simulink model "Quadcopter_2DoF_Model_7_b"  (R2025b)
settings: Solver=ode23t  StartTime=0.0  StopTime=T_mis  FixedStep=0.02  MaxStep=0.001  RelTol=1e-3
InitFcn:
  | % Make sure MATLAB can find the model folder and the battery data folder
  | modelDir = fileparts(get_param(bdroot, 'FileName'));
  | addpath(modelDir);  % finds mission_config.m
  | addpath(fullfile(modelDir, '..', 'Battery_data', 'output')); % finds hppc_params.mat
  | 
  | 
  | %Quadcopter parameters
  | Jyy = 5.343596e-5; %Mass moment of inertia about yB(kg.m^2)
  | Jxx = 5.473766e-5;%Mass moment of inertia about xB(kg.m^2)
  | Jzz = 9.8934e-5;%Mass moment of inertia about zB(kg.m^2)
  | m = 0.1207; %Total mass of the quadcopter (kg)
  | g = 9.81; %gravitational acceleration
  | k_f = 7.22e-8; %thrust coefficient
  | k_tau = 5.11e-10; %torque coefficient. smaller than kf
  | l = 0.05433; %Arm length, COM to each motor shaft
  | 
  | %Battery parameters
  | if ~exist('soc0', 'var'), soc0 = 1; end
  | load('hppc_params.mat', 'soc_grid', 'tables');
  | 
  | idx      = 1:5:101; % every 5% SOC, 21 points
  | SOC_vec  = soc_grid(idx)'; % 0, 0.05, ... 1
  | V0_vec   = tables.OCV(idx)';
  | R0_vec   = tables.R0(idx)'  / 1000;
  | R1_vec   = tables.R1(idx)'  / 1000;
  | tau1_vec = R1_vec .* tables.C1(idx)';
  | 
  | %Mission parameters
  | mis = mission_config('fast_move', false);
  | t_mis = mis.t;
  | z_ref = mis.z;
  | x_ref = mis.x;
  | T_mis = mis.T;
values from neighbouring files (symbols this model uses):
  soc_grid = [0 0.01 0.02 0.03 0.04 0.05 0.06 0.07 0.08 0.09 0.1 0.11 ... (101 elements, 101x1)]    [hppc_params.mat]
  tables =     [hppc_params.mat]
libraries: fl_lib x4, slpidlib x3, nesl_utility x3, simulink x3
settings Model: Creator=Haaniya  LastModifiedBy=Haaniya
settings DataIOCC: ReturnWorkspaceOutputs=off

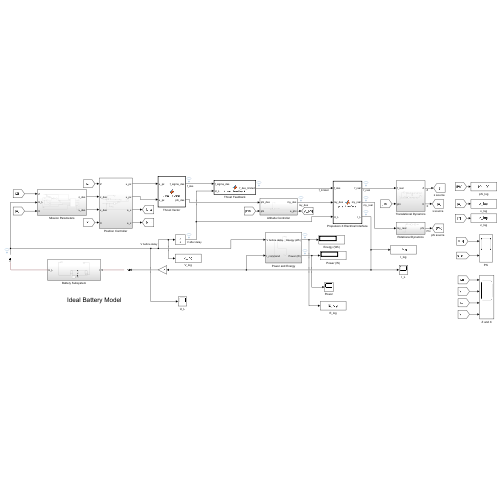
[thumbnail: Simulink's stored preview of the top-level diagram]
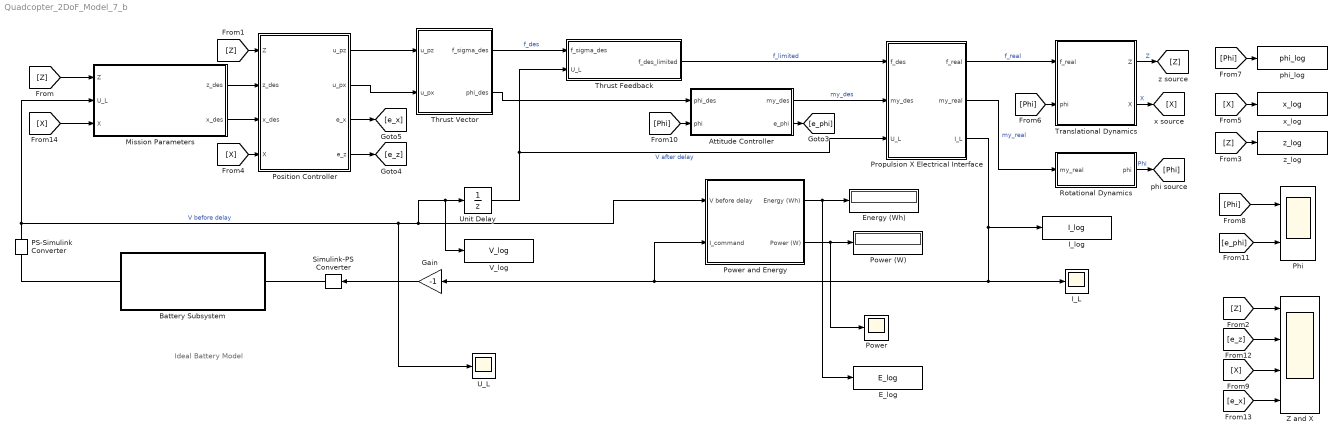
== system Quadcopter_2DoF_Model_7_b ==
  note: Ideal Battery Model
  Attitude Controller : Subsystem
  Battery Subsystem : Subsystem
  E_log : ToWorkspace  VariableName=E_log  SaveFormat=Timeseries  SampleTime=-1
  Energy (Wh) : Display
  Gain : Gain  Gain=-1
  I_L : Scope
      settings: ActiveDisplayYMinimum=-1  ActiveDisplayYMaximum=1  DataLoggingVariableName=ScopeData5
  I_log : ToWorkspace  VariableName=I_log  SaveFormat=Timeseries  SampleTime=-1
  Mission Parameters : Subsystem
  PS-Simulink Converter : nesl_utility/PS-Simulink Converter  PhysicalDomain=network_engine_domain  SubClassName=ps_output  LeftPortType=input  RightPortType=output  PseudoPeriodic=off  Frequencies=[]  VectorFormat=inherit  Unit=inherit  AffineConversion=off
  Phi : Scope  NumInputPorts=2
      settings: ActiveDisplayYMinimum=-0.256680900083002  ActiveDisplayYMaximum=0.30893996648524746
  Position Controller : Subsystem
  Power : Scope
      settings: ActiveDisplayYMinimum=-1  ActiveDisplayYMaximum=1
  Power (W) : Display
  Power and Energy : Subsystem
  Propulsion X Electrical Interface : MATLAB Function  TreatAsAtomicUnit=on
  Rotational Dynamics : Subsystem
  Simulink-PS Converter : nesl_utility/Simulink-PS Converter  PhysicalDomain=network_engine_domain  SubClassName=ps_input  LeftPortType=input  RightPortType=output  PseudoPeriodic=off  Frequencies=[]  NoiseDistribution=none  NoiseParameters=[]  Unit=1  AffineConversion=off  FilteringAndDerivatives=provide  SimscapeFilterOrder=1  InputFilterTimeConstant=0.001  UdotUserProvided=0
  Thrust Feedback : MATLAB Function  TreatAsAtomicUnit=on
  Thrust Vector : MATLAB Function  TreatAsAtomicUnit=on
  Translational Dynamics : Subsystem
  U_L : Scope
      settings: ActiveDisplayYMinimum=-1  ActiveDisplayYMaximum=1  DataLoggingVariableName=ScopeData4
  Unit Delay : UnitDelay  InitialCondition=12.6  SampleTime=-1  HasFrameUpgradeWarning=on
  V_log : ToWorkspace  VariableName=V_log  SaveFormat=Timeseries  SampleTime=-1
  Z and X : Scope  NumInputPorts=4
      settings: ActiveDisplayYMinimum=-2.8823289084594785  ActiveDisplayYMaximum=7.6709964500964789  DataLoggingVariableName=ScopeData2
  phi_log : ToWorkspace  VariableName=phi_log  SaveFormat=Timeseries  SampleTime=0.02
  x_log : ToWorkspace  VariableName=x_log  SaveFormat=Timeseries  SampleTime=0.02
  z_log : ToWorkspace  VariableName=z_log  SaveFormat=Timeseries  SampleTime=0.02
  wires:
  Position Controller/2(u_px) -> Thrust Vector/2(u_px)
  Position Controller/1(u_pz) -> Thrust Vector/1(u_pz)
  Thrust Vector/2(phi_des) -> Attitude Controller/1(phi_des)
  Propulsion X Electrical Interface/2(my_real) -> Rotational Dynamics/1(my_real)  "my_real"
  Unit Delay/1 -> Thrust Feedback/2(U_L), Propulsion X Electrical Interface/3(U_L)  "V after delay"
  PS-Simulink Converter/1 -> Mission Parameters/2(U_L), U_L/1, V_log/1, Unit Delay/1, Power and Energy/1(V before delay)  "V before delay"
  Gain/1 -> Simulink-PS Converter/1
  Propulsion X Electrical Interface/3(I_L) -> I_L/1, Power and Energy/2(I_command), Gain/1, I_log/1
  Propulsion X Electrical Interface/1(f_real) -> Translational Dynamics/1(f_real)  "f_real"
  Attitude Controller/1(my_des) -> Propulsion X Electrical Interface/2(my_des)  "my_des"
  Thrust Vector/1(f_sigma_des) -> Thrust Feedback/1(f_sigma_des)  "f_des"
  Thrust Feedback/1(f_des_limited) -> Propulsion X Electrical Interface/1(f_des)  "f_limited"
  Mission Parameters/1(z_des) -> Position Controller/2(z_des)
  Mission Parameters/2(x_des) -> Position Controller/3(x_des)
  [Z] -> Mission Parameters/1(Z)
  [Z] -> Position Controller/1(Z)
  [Z] -> Z and X/1
  Translational Dynamics/1(Z) -> [Z]  "Z"
  [Z] -> z_log/1
  [X] -> Position Controller/4(X)
  [X] -> x_log/1
  Translational Dynamics/2(X) -> [X]  "X"
  [Phi] -> Translational Dynamics/2(phi)
  [Phi] -> phi_log/1
  [Phi] -> Phi/1
  [X] -> Z and X/3
  [Phi] -> Attitude Controller/2(phi)
  Rotational Dynamics/1(phi) -> [Phi]  "Phi"
  [e_phi] -> Phi/2
  [e_z] -> Z and X/2
  [e_x] -> Z and X/4
  Attitude Controller/2(e_phi) -> [e_phi]
  Position Controller/4(e_z) -> [e_z]
  Position Controller/3(e_x) -> [e_x]
  Power and Energy/1(Energy (Wh)) -> E_log/1, Energy (Wh)/1
  Power and Energy/2(Power (W)) -> Power/1, Power (W)/1
  [X] -> Mission Parameters/3(X)
  connections:
  Battery Subsystem/LConn1 -- PS-Simulink Converter/LConn1
  Simulink-PS Converter/RConn1 -- Battery Subsystem/RConn1

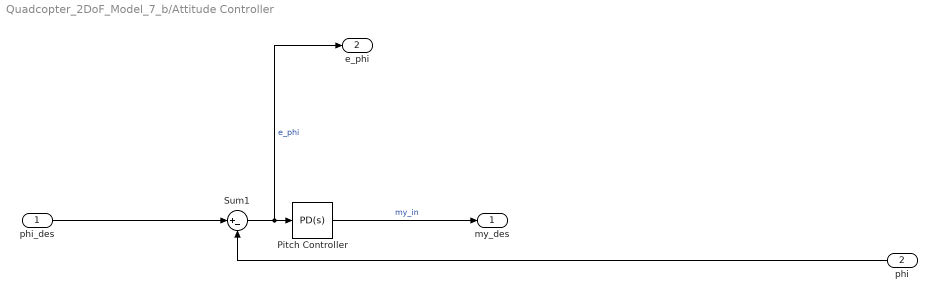
== system Quadcopter_2DoF_Model_7_b/Attitude Controller ==
  phi_des : Inport
  phi : Inport  Port=2
  Pitch Controller : slpidlib/PID Controller  Controller=PD  Form=Parallel  TimeDomain=Continuous-time  UseExternalTs=off  SampleTime=-1  IntegratorMethod=Forward Euler  FilterMethod=Forward Euler  ControllerParametersSource=internal  P=0.000320082486755336  I=1  UseKiTs=off  D=0.000451023727668426  UseExternalDerivativeSource=off  N=23.8205218545542  UseFilter=on  TunerSelectOption=Transfer Function Based (PID Tuner App)  InitialConditionSource=internal  InitialConditionForIntegrator=0  InitialConditionForFilter=0  DifferentiatorICPrevScaledInput=0  ExternalReset=none  TrackingMode=off  Kt=1  LimitOutput=off  SatLimitsSource=internal  UpperSaturationLimit=inf  LowerSaturationLimit=-inf  LinearizeAsGain=on  AntiWindupMode=none  Kb=1  LimitIntegrator=off  UpperIntegratorSaturationLimit=inf  LowerIntegratorSaturationLimit=-inf  POutMin=[]  POutMax=[]  IOutMin=[]  IOutMax=[]  DOutMin=[]  DOutMax=[]  NOutMin=[]  NOutMax=[]  SumOutMin=[]  SumOutMax=[]  SaturationOutMin=[]  SaturationOutMax=[]  PParamMin=[]  PParamMax=[]  IParamMin=[]  IParamMax=[]  DParamMin=[]  DParamMax=[]  NParamMin=[]  NParamMax=[]  KbParamMin=[]  KbParamMax=[]  KtParamMin=[]  KtParamMax=[]  KbOutMin=[]  KbOutMax=[]  KtOutMin=[]  KtOutMax=[]  IntegratorOutMin=[]  IntegratorOutMax=[]  FilterOutMin=[]  FilterOutMax=[]  SumI1OutMin=[]  SumI1OutMax=[]  SumI2OutMin=[]  SumI2OutMax=[]  SumI3OutMin=[]  SumI3OutMax=[]  SumI4OutMin=[]  SumI4OutMax=[]  SumDOutMin=[]  SumDOutMax=[]  DifferentiatorOutMin=[]  DifferentiatorOutMax=[]  FilterDiffOutCoefMin=[]  FilterDiffOutCoefMax=[]  ReciprocalOutMin=[]  ReciprocalOutMax=[]  SumDenOutMin=[]  SumDenOutMax=[]  SumNumOutMin=[]  SumNumOutMax=[]  DivideOutMin=[]  DivideOutMax=[]  UdiffTsProdOutMin=[]  UdiffTsProdOutMax=[]  NTsProdOutMin=[]  NTsProdOutMax=[]  UintegralTsProdOutMin=[]  UintegralTsProdOutMax=[]  UngainTsProdOutMin=[]  UngainTsProdOutMax=[]  ClampingZeroOutDataTypeStr=Inherit: Inherit via back propagation  ClampingZeroOutMin=[]  ClampingZeroOutMax=[]  FilterDenConstantOutDataTypeStr=Inherit: Inherit via back propagation  FilterDenConstantOutMin=[]  FilterDenConstantOutMax=[]  PCopyOutDataTypeStr=Inherit: Inherit via back propagation  PCopyOutMin=[]  PCopyOutMax=[]  NCopyOutDataTypeStr=Inherit: Inherit via back propagation  NCopyOutMin=[]  NCopyOutMax=[]  IntegratorContinuousStateAttributes=''  IntegratorStateMustResolveToSignalObject=off  IntegratorRTWStateStorageClass=Auto  FilterContinuousStateAttributes=''  FilterStateMustResolveToSignalObject=off  FilterRTWStateStorageClass=Auto  ParallelPVariant=InternalParameters  IdealPVariant=Disabled  IVariant=Disabled  DVariant=InternalParameters  IntegratorVariant=Disabled  SatVariant=Disabled  AWVariant=Disabled  PCopyVariant=Disabled  TRVariant=Disabled  FdbkBlocksVariant=Forward  IdealPFdbkVariant=Disabled  SatFdbkVariant=Disabled  DerivativeFilterVariant=ContFilter  NVariant=InternalParameters  NCopyVariant=Disabled  FilterICVariant=InternalICsFilter  IntegratorICVariant=Disabled  ExternalResetVariant=Disabled  TRSumVariant=Passthrough  SumFdbkVariant=Disabled  SumVariant=Sum_PD  TsampFilterVariant=InternalTs  TsampNgainVariant=Passthrough  TsampIntegralVariant=Disabled_SignalSpec  ExternalSaturationOutDataTypeStr=Inherit: Same as second input  DerivativeSourceVariant=ErrorSignal  PreIntVariant=InternalPreInt
  Sum1 : Sum  Inputs=|+-
  my_des : Outport
  e_phi : Outport  Port=2
  wires:
  Sum1/1 -> e_phi/1, Pitch Controller/1  "e_phi"
  phi/1 -> Sum1/2
  Pitch Controller/1 -> my_des/1  "my_in"
  phi_des/1 -> Sum1/1

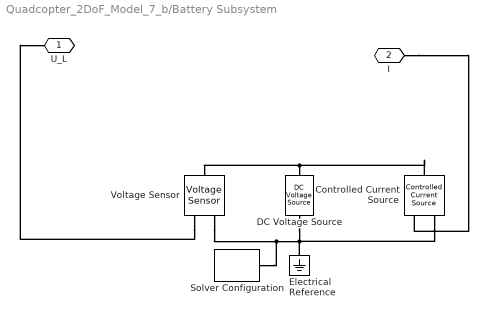
== system Quadcopter_2DoF_Model_7_b/Battery Subsystem ==
  Controlled Current Source : fl_lib/Electrical/Electrical Sources/Controlled Current Source
  DC Voltage Source : fl_lib/Electrical/Electrical Sources/DC Voltage Source  v0=12.6 V
  Electrical Reference : fl_lib/Electrical/Electrical Elements/Electrical Reference
  Solver Configuration : nesl_utility/Solver Configuration  PhysicalDomain=network_engine_domain  SubClassName=solver  LeftPortType=input  RightPortType=generic  Tones=[]  Harmonics=[]  SimulateNoise=off  Profile=off  UseLocalSampling=off  EnableSwitchedLinearOptims=on  FrequencyDomain=off  UseCCode=off  RelTol=0.001  AbsTol=0.001  MinStep=1e-09  ToWorkspace=off  RevertToSquareIcSolve=off  NumHomotopyIterations=100  PhasorMode=off  PhasorModeNumHarmonics=1  ConsistencySolver=NEWTON_XTOL_AFTER_FTOL  IndexReductionMethod=DerivativeReplacement  DoDC=off  ResidualTolerance=1e-09  ConsistencyTolSource=GLOBAL  ConsistencyAbsTol=0.001  ConsistencyRelTol=0.001  ConsistencyTolFactor=0.001  UseLocalSolver=off  LocalSolverChoice=NE_BACKWARD_EULER_ADVANCER  ResolveIndetEquations=on  FunctionEvalNumThread=1  LocalSolverSampleTime=0.001  DoFixedCost=off  MaxNonlinIter=3  MaxModeIter=2  ComputeImpulses=off  ImpulseIterations=2  LinearAlgebra=auto  LinearAlgebraNumThread=0  EquationFormulation=NE_TIME_EF  DelaysMemoryBudget=1024  AutomaticFiltering=on  FilteringTimeConstant=0.001  PartitionStorageMethod=AS_NEEDED  PartitionMemoryBudget=1024  PartitionMethod=ROBUST  MultibodyUseLocalSolver=off  MultibodyLocalSolverChoice=ODE1  MultibodyLocalSolverSampleTime=0.001
  Voltage Sensor : fl_lib/Electrical/Electrical Sensors/Voltage Sensor
  U_L : PMIOPort  Side=Left
  I : PMIOPort  Port=2  Side=Right
  connections:
  I/RConn1 -- Controlled Current Source/RConn1
  Voltage Sensor/RConn2 -- DC Voltage Source/RConn1 -- Electrical Reference/LConn1 -- Controlled Current Source/RConn2 -- Solver Configuration/RConn1
  Controlled Current Source/LConn1 -- DC Voltage Source/LConn1 -- Voltage Sensor/LConn1
  Voltage Sensor/RConn1 -- U_L/RConn1

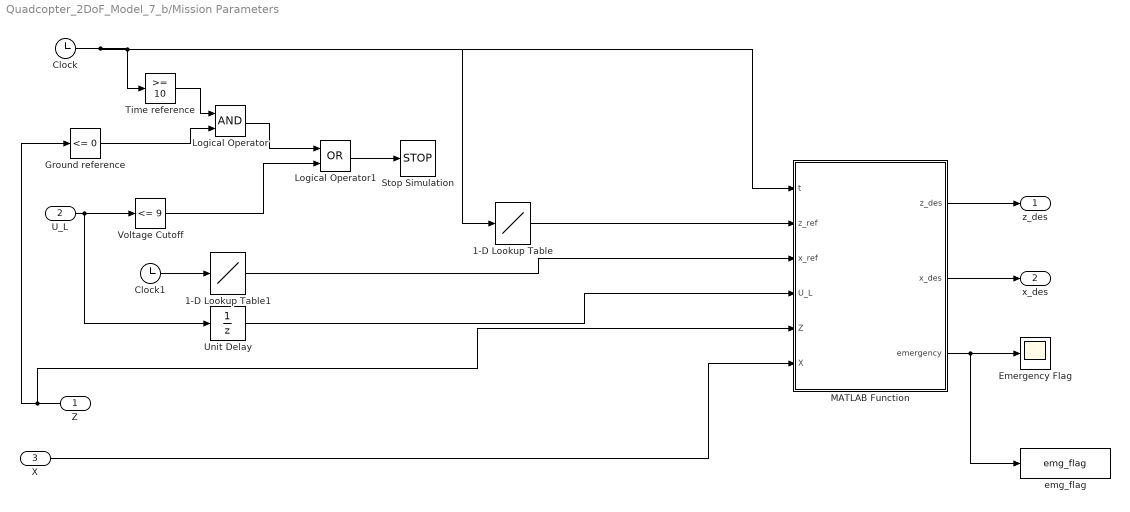
== system Quadcopter_2DoF_Model_7_b/Mission Parameters ==
  Z : Inport
  U_L : Inport  Port=2
  X : Inport  Port=3
  1-D Lookup Table : Lookup_n-D  NumberOfTableDimensions=1  BreakpointsForDimension1=t_mis  Table=z_ref  InternalRulePriority=Speed  RndMeth=Simplest
  1-D Lookup Table1 : Lookup_n-D  NumberOfTableDimensions=1  BreakpointsForDimension1=t_mis  Table=x_ref  InternalRulePriority=Speed  RndMeth=Simplest
  Clock : Clock
  Clock1 : Clock
  "Emergency Flag " : Scope
      settings: ActiveDisplayYMinimum=0.37624445803361362  ActiveDisplayYMaximum=1.0722912307555632  DataLoggingVariableName=ScopeData6
  Ground reference : simulink/Logic and Bit Operations/Compare To Constant  relop=<=  const=0  OutDataTypeStr=boolean
  Logical Operator : Logic  AllPortsSameDT=off  OutDataTypeStr=boolean
  Logical Operator1 : Logic  Operator=OR  AllPortsSameDT=off  OutDataTypeStr=boolean
  MATLAB Function : MATLAB Function  TreatAsAtomicUnit=on
  Stop Simulation : Stop
  Time reference : simulink/Logic and Bit Operations/Compare To Constant  relop=>=  const=10  OutDataTypeStr=boolean
  Unit Delay : UnitDelay  SampleTime=-1  HasFrameUpgradeWarning=on
  Voltage Cutoff : simulink/Logic and Bit Operations/Compare To Constant  relop=<=  const=9  OutDataTypeStr=boolean
  emg_flag : ToWorkspace  VariableName=emg_flag  SaveFormat=Timeseries  SampleTime=-1
  z_des : Outport
  x_des : Outport  Port=2
  wires:
  Clock/1 -> MATLAB Function/1(t), Time reference/1, 1-D Lookup Table/1
  Z/1 -> MATLAB Function/5(Z), Ground reference/1
  1-D Lookup Table/1 -> MATLAB Function/2(z_ref)
  Time reference/1 -> Logical Operator/1
  Clock1/1 -> 1-D Lookup Table1/1
  Ground reference/1 -> Logical Operator/2
  Logical Operator1/1 -> Stop Simulation/1
  Logical Operator/1 -> Logical Operator1/1
  Voltage Cutoff/1 -> Logical Operator1/2
  U_L/1 -> Unit Delay/1, Voltage Cutoff/1
  MATLAB Function/1(z_des) -> z_des/1
  MATLAB Function/2(x_des) -> x_des/1
  1-D Lookup Table1/1 -> MATLAB Function/3(x_ref)
  X/1 -> MATLAB Function/6(X)
  MATLAB Function/3(emergency) -> emg_flag/1, "Emergency Flag "/1
  Unit Delay/1 -> MATLAB Function/4(U_L)

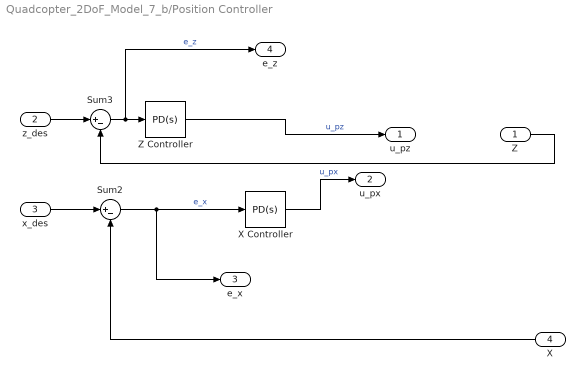
== system Quadcopter_2DoF_Model_7_b/Position Controller ==
  Z : Inport
  z_des : Inport  Port=2
  x_des : Inport  Port=3
  X : Inport  Port=4
  Sum2 : Sum  Inputs=|+-
  Sum3 : Sum  Inputs=|+-
  X Controller : slpidlib/PID Controller  Controller=PD  Form=Parallel  TimeDomain=Continuous-time  UseExternalTs=off  SampleTime=-1  IntegratorMethod=Forward Euler  FilterMethod=Forward Euler  ControllerParametersSource=internal  P=0.0253006074053555  I=1  UseKiTs=off  D=0.117802026720809  UseExternalDerivativeSource=off  N=10  UseFilter=on  TunerSelectOption=Transfer Function Based (PID Tuner App)  InitialConditionSource=internal  InitialConditionForIntegrator=0  InitialConditionForFilter=0  DifferentiatorICPrevScaledInput=0  ExternalReset=none  TrackingMode=off  Kt=1  LimitOutput=off  SatLimitsSource=internal  UpperSaturationLimit=inf  LowerSaturationLimit=-inf  LinearizeAsGain=on  AntiWindupMode=none  Kb=1  LimitIntegrator=off  UpperIntegratorSaturationLimit=inf  LowerIntegratorSaturationLimit=-inf  POutMin=[]  POutMax=[]  IOutMin=[]  IOutMax=[]  DOutMin=[]  DOutMax=[]  NOutMin=[]  NOutMax=[]  SumOutMin=[]  SumOutMax=[]  SaturationOutMin=[]  SaturationOutMax=[]  PParamMin=[]  PParamMax=[]  IParamMin=[]  IParamMax=[]  DParamMin=[]  DParamMax=[]  NParamMin=[]  NParamMax=[]  KbParamMin=[]  KbParamMax=[]  KtParamMin=[]  KtParamMax=[]  KbOutMin=[]  KbOutMax=[]  KtOutMin=[]  KtOutMax=[]  IntegratorOutMin=[]  IntegratorOutMax=[]  FilterOutMin=[]  FilterOutMax=[]  SumI1OutMin=[]  SumI1OutMax=[]  SumI2OutMin=[]  SumI2OutMax=[]  SumI3OutMin=[]  SumI3OutMax=[]  SumI4OutMin=[]  SumI4OutMax=[]  SumDOutMin=[]  SumDOutMax=[]  DifferentiatorOutMin=[]  DifferentiatorOutMax=[]  FilterDiffOutCoefMin=[]  FilterDiffOutCoefMax=[]  ReciprocalOutMin=[]  ReciprocalOutMax=[]  SumDenOutMin=[]  SumDenOutMax=[]  SumNumOutMin=[]  SumNumOutMax=[]  DivideOutMin=[]  DivideOutMax=[]  UdiffTsProdOutMin=[]  UdiffTsProdOutMax=[]  NTsProdOutMin=[]  NTsProdOutMax=[]  UintegralTsProdOutMin=[]  UintegralTsProdOutMax=[]  UngainTsProdOutMin=[]  UngainTsProdOutMax=[]  ClampingZeroOutDataTypeStr=Inherit: Inherit via back propagation  ClampingZeroOutMin=[]  ClampingZeroOutMax=[]  FilterDenConstantOutDataTypeStr=Inherit: Inherit via back propagation  FilterDenConstantOutMin=[]  FilterDenConstantOutMax=[]  PCopyOutDataTypeStr=Inherit: Inherit via back propagation  PCopyOutMin=[]  PCopyOutMax=[]  NCopyOutDataTypeStr=Inherit: Inherit via back propagation  NCopyOutMin=[]  NCopyOutMax=[]  IntegratorContinuousStateAttributes=''  IntegratorStateMustResolveToSignalObject=off  IntegratorRTWStateStorageClass=Auto  FilterContinuousStateAttributes=''  FilterStateMustResolveToSignalObject=off  FilterRTWStateStorageClass=Auto  ParallelPVariant=InternalParameters  IdealPVariant=Disabled  IVariant=Disabled  DVariant=InternalParameters  IntegratorVariant=Disabled  SatVariant=Disabled  AWVariant=Disabled  PCopyVariant=Disabled  TRVariant=Disabled  FdbkBlocksVariant=Forward  IdealPFdbkVariant=Disabled  SatFdbkVariant=Disabled  DerivativeFilterVariant=ContFilter  NVariant=InternalParameters  NCopyVariant=Disabled  FilterICVariant=InternalICsFilter  IntegratorICVariant=Disabled  ExternalResetVariant=Disabled  TRSumVariant=Passthrough  SumFdbkVariant=Disabled  SumVariant=Sum_PD  TsampFilterVariant=InternalTs  TsampNgainVariant=Passthrough  TsampIntegralVariant=Disabled_SignalSpec  ExternalSaturationOutDataTypeStr=Inherit: Same as second input  DerivativeSourceVariant=ErrorSignal  PreIntVariant=InternalPreInt
  Z Controller : slpidlib/PID Controller  Controller=PD  Form=Parallel  TimeDomain=Continuous-time  UseExternalTs=off  SampleTime=-1  IntegratorMethod=Forward Euler  FilterMethod=Forward Euler  ControllerParametersSource=internal  P=0.0253006074053555  I=1  UseKiTs=off  D=0.117802026720809  UseExternalDerivativeSource=off  N=10  UseFilter=on  TunerSelectOption=Transfer Function Based (PID Tuner App)  InitialConditionSource=internal  InitialConditionForIntegrator=0  InitialConditionForFilter=0  DifferentiatorICPrevScaledInput=0  ExternalReset=none  TrackingMode=off  Kt=1  LimitOutput=off  SatLimitsSource=internal  UpperSaturationLimit=inf  LowerSaturationLimit=-inf  LinearizeAsGain=on  AntiWindupMode=none  Kb=1  LimitIntegrator=off  UpperIntegratorSaturationLimit=inf  LowerIntegratorSaturationLimit=-inf  POutMin=[]  POutMax=[]  IOutMin=[]  IOutMax=[]  DOutMin=[]  DOutMax=[]  NOutMin=[]  NOutMax=[]  SumOutMin=[]  SumOutMax=[]  SaturationOutMin=[]  SaturationOutMax=[]  PParamMin=[]  PParamMax=[]  IParamMin=[]  IParamMax=[]  DParamMin=[]  DParamMax=[]  NParamMin=[]  NParamMax=[]  KbParamMin=[]  KbParamMax=[]  KtParamMin=[]  KtParamMax=[]  KbOutMin=[]  KbOutMax=[]  KtOutMin=[]  KtOutMax=[]  IntegratorOutMin=[]  IntegratorOutMax=[]  FilterOutMin=[]  FilterOutMax=[]  SumI1OutMin=[]  SumI1OutMax=[]  SumI2OutMin=[]  SumI2OutMax=[]  SumI3OutMin=[]  SumI3OutMax=[]  SumI4OutMin=[]  SumI4OutMax=[]  SumDOutMin=[]  SumDOutMax=[]  DifferentiatorOutMin=[]  DifferentiatorOutMax=[]  FilterDiffOutCoefMin=[]  FilterDiffOutCoefMax=[]  ReciprocalOutMin=[]  ReciprocalOutMax=[]  SumDenOutMin=[]  SumDenOutMax=[]  SumNumOutMin=[]  SumNumOutMax=[]  DivideOutMin=[]  DivideOutMax=[]  UdiffTsProdOutMin=[]  UdiffTsProdOutMax=[]  NTsProdOutMin=[]  NTsProdOutMax=[]  UintegralTsProdOutMin=[]  UintegralTsProdOutMax=[]  UngainTsProdOutMin=[]  UngainTsProdOutMax=[]  ClampingZeroOutDataTypeStr=Inherit: Inherit via back propagation  ClampingZeroOutMin=[]  ClampingZeroOutMax=[]  FilterDenConstantOutDataTypeStr=Inherit: Inherit via back propagation  FilterDenConstantOutMin=[]  FilterDenConstantOutMax=[]  PCopyOutDataTypeStr=Inherit: Inherit via back propagation  PCopyOutMin=[]  PCopyOutMax=[]  NCopyOutDataTypeStr=Inherit: Inherit via back propagation  NCopyOutMin=[]  NCopyOutMax=[]  IntegratorContinuousStateAttributes=''  IntegratorStateMustResolveToSignalObject=off  IntegratorRTWStateStorageClass=Auto  FilterContinuousStateAttributes=''  FilterStateMustResolveToSignalObject=off  FilterRTWStateStorageClass=Auto  ParallelPVariant=InternalParameters  IdealPVariant=Disabled  IVariant=Disabled  DVariant=InternalParameters  IntegratorVariant=Disabled  SatVariant=Disabled  AWVariant=Disabled  PCopyVariant=Disabled  TRVariant=Disabled  FdbkBlocksVariant=Forward  IdealPFdbkVariant=Disabled  SatFdbkVariant=Disabled  DerivativeFilterVariant=ContFilter  NVariant=InternalParameters  NCopyVariant=Disabled  FilterICVariant=InternalICsFilter  IntegratorICVariant=Disabled  ExternalResetVariant=Disabled  TRSumVariant=Passthrough  SumFdbkVariant=Disabled  SumVariant=Sum_PD  TsampFilterVariant=InternalTs  TsampNgainVariant=Passthrough  TsampIntegralVariant=Disabled_SignalSpec  ExternalSaturationOutDataTypeStr=Inherit: Same as second input  DerivativeSourceVariant=ErrorSignal  PreIntVariant=InternalPreInt
  u_pz : Outport
  u_px : Outport  Port=2
  e_x : Outport  Port=3
  e_z : Outport  Port=4
  wires:
  X/1 -> Sum2/2
  Z/1 -> Sum3/2
  z_des/1 -> Sum3/1
  Sum2/1 -> e_x/1, X Controller/1  "e_x"
  Sum3/1 -> e_z/1, Z Controller/1  "e_z"
  x_des/1 -> Sum2/1
  X Controller/1 -> u_px/1  "u_px"
  Z Controller/1 -> u_pz/1  "u_pz"

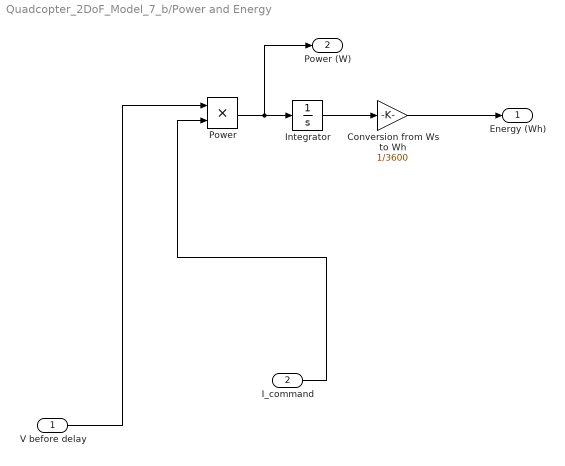
== system Quadcopter_2DoF_Model_7_b/Power and Energy ==
  V before delay : Inport
  I_command : Inport  Port=2
  Conversion from Ws to Wh : Gain  Gain=1/3600
  Integrator : Integrator
  Power : Product
  Energy (Wh) : Outport
  Power (W) : Outport  Port=2
  wires:
  Conversion from Ws to Wh/1 -> Energy (Wh)/1
  Integrator/1 -> Conversion from Ws to Wh/1
  Power/1 -> Power (W)/1, Integrator/1
  V before delay/1 -> Power/1
  I_command/1 -> Power/2

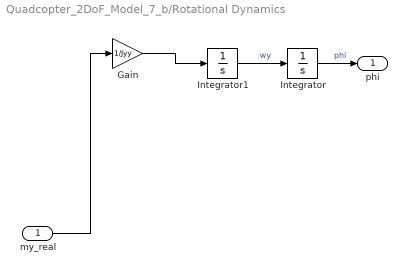
== system Quadcopter_2DoF_Model_7_b/Rotational Dynamics ==
  my_real : Inport
  Gain : Gain  Gain=1/Jyy
  Integrator : Integrator
  Integrator1 : Integrator
  phi : Outport
  wires:
  Integrator1/1 -> Integrator/1  "wy"
  Gain/1 -> Integrator1/1
  my_real/1 -> Gain/1
  Integrator/1 -> phi/1  "phi"

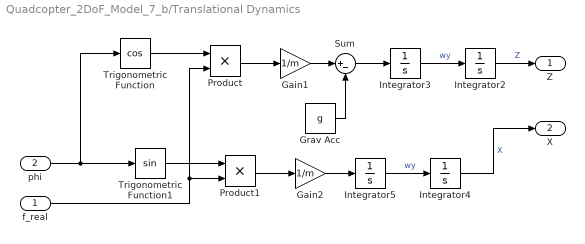
== system Quadcopter_2DoF_Model_7_b/Translational Dynamics ==
  f_real : Inport
  phi : Inport  Port=2
  Gain1 : Gain  Gain=1/m
  Gain2 : Gain  Gain=1/m
  Grav Acc : Constant  Value=g
  Integrator{2..5} (4 alike) : Integrator
  Product : Product
  Product1 : Product
  Sum : Sum  Inputs=|+-
  Trigonometric Function : Trigonometry  Operator=cos
  Trigonometric Function1 : Trigonometry
  Z : Outport
  X : Outport  Port=2
  wires:
  Grav Acc/1 -> Sum/2
  Trigonometric Function1/1 -> Product1/1
  phi/1 -> Trigonometric Function/1, Trigonometric Function1/1
  Product1/1 -> Gain2/1
  Sum/1 -> Integrator3/1
  Product/1 -> Gain1/1
  Gain1/1 -> Sum/1
  Trigonometric Function/1 -> Product/1
  Integrator2/1 -> Z/1  "Z"
  f_real/1 -> Product1/2, Product/2
  Gain2/1 -> Integrator5/1
  Integrator3/1 -> Integrator2/1  "wy"
  Integrator5/1 -> Integrator4/1  "wy"
  Integrator4/1 -> X/1  "X"

== matlab function Quadcopter_2DoF_Model_7_b/Thrust Vector ==
  data: u_pz input; u_px input; f_sigma_des output; phi_des output
function [f_sigma_des, phi_des] = thrust_vector(u_pz, u_px)

m =0.1207;
g = 9.81;

Fx= u_px;
Fz= u_pz+m*g;

f_sigma_des = sqrt(Fx^2+Fz^2);

phi_des = atan2(Fx, Fz);

end

== matlab function Quadcopter_2DoF_Model_7_b/Mission Parameters/MATLAB Function ==
  settings: updateMethod=DISCRETE
  data: t input; z_des output; z_ref input; x_ref input; U_L input; Z input; X input; x_des output; emergency output
function [z_des, x_des, emergency] = emergency_stop(t, z_ref, x_ref, U_L, Z, X)

V_trig = 9.6; %3.2V per cell
v_land = 0.8; % emergency landing speed

persistent triggered t0 z0 x0
if isempty(triggered)
    triggered= false; 
    t0=0; 
    z0=0;
    x0=0;
end


if ~triggered && t>10 && U_L<V_trig %if triggered, take note of where triggered 
    % and continue staying triggered
    triggered = true;
    t0 = t;
    z0 = Z;
    x0 = X;
end

if triggered
    z_des = max(z0 - v_land*(t-t0), 0);%ramp down
    x_des = x0;%hold horizontal pos
else
    z_des = z_ref;%if not triggered then continue with normal position
    x_des =x_ref;
end

emergency = double(triggered);%indicator which is 1 once active

end

== matlab function Quadcopter_2DoF_Model_7_b/Propulsion X Electrical Interface ==
  data: f_real output; my_real output; I_L output; f_des input; my_des input; U_L input
function [f_real, my_real, I_L] = p_e_interface(f_des, my_des,U_L)

%Constants:
k_f = 7.22e-8; %thrust coefficient 
k_tau = 5.11e-10; %torque coefficient. smaller than kf
l = 0.05433; %Arm length, COM to each motor shaft
Kv_rad = 7047*(2*pi/60);
Kt = 1/Kv_rad; % torque constant, from fitted Kv_rad
R_int = 0.586;

%inverted motor mixing - formulae taken from notes
%given total desired thrust and pitch moment -> individual rotor thrusts
f1_cmd = f_des/4 - my_des/(2*l);
f3_cmd = f_des/4 + my_des/(2*l);
f24_cmd = f_des/4; %no pitch contribution because only working in zx plane

%rotors have a minimum of zero. Negative thrust is unphysical because rotors
%cannot spin backward to produce a negative thrust
f1_cmd = max(f1_cmd, 0);
f3_cmd = max(f3_cmd, 0);
f24_cmd = max(f24_cmd, 0);

%inverts using f=kf*w formula. Speed the controller is asking for
w1_cmd =sqrt(f1_cmd/k_f);
w3_cmd =sqrt(f3_cmd/k_f);
w24_cmd = sqrt((f_des/4)/k_f);

%Quadratic from motor voltage balance equation where solves for fastest any
%rotor can spin at current battery voltage
%Same value for all 4 rotors, since they share a motor type and a battery

a = R_int*k_tau/Kt;
b = Kt;
c = -U_L;
w_max = (-b +sqrt(b^2-4*a*c))/(2*a);

% Saturation: triggers when either w1 or w3 exceeds maximum speed

d = abs(w3_cmd^2 - w1_cmd^2);

if max(w1_cmd, w3_cmd)>w_max
    w_hi =w_max;
    w_lo =sqrt(max(w_max^2-d,0));
    if w3_cmd >= w1_cmd
        w3 =w_hi; w1= w_lo;
    else
        w1 = w_hi; w3 =w_lo;
    end
else
    w1 =w1_cmd; w3 = w3_cmd;

end

w24 = min(w24_cmd, w_max);

%recompute actual thrust and moment
f1_real = k_f*w1^2;
f3_real = k_f*w3^2;
f24_real = k_f*w24^2;

f_real = f1_real+f3_real+2*f24_real;
my_real = l*(f3_real-f1_real);

%current draw
tau1 = k_tau*w1^2;
tau3 = k_tau*w3^2;

I1 = tau1/Kt;
I3 = tau3/Kt;
I24 = (k_tau*w24^2)/Kt;
I_L = I1+I3+2*I24;

end

== matlab function Quadcopter_2DoF_Model_7_b/Thrust Feedback ==
  data: f_sigma_des input; f_des_limited output; U_L input
function f_des_limited  = thrust_feedback(f_sigma_des, U_L)

k_f = 7.22e-8; %thrust coefficient 
k_tau = 5.11e-10; %torque coefficient. smaller than kf
Kv_rad = 7047*(2*pi/60);
Kt = 1/Kv_rad; % torque constant, from fitted Kv_rad
R_int = 0.586;

a = R_int*k_tau/Kt;
b = Kt; 
c = -U_L;

w_max = (-b +sqrt(b^2-4*a*c))/(2*a);

f_max = 4*k_f*w_max^2;
f_des_limited = min(f_sigma_des, f_max);

end
